simulink model "drone_yolo_simulasyon"  (R2025b)
settings: Solver=VariableStepAuto  StartTime=0.0  StopTime=15.0  RelTol=1e-3
undefined symbols (not defined in the file): Sim3dSensor
libraries: visionsources x1, pycoexlib x1, visiongeotforms x1, sim3dcameralib x1, sim3dlib x1, uavsim3dlib x1
settings Model: Creator=sario  LastModifiedBy=sario

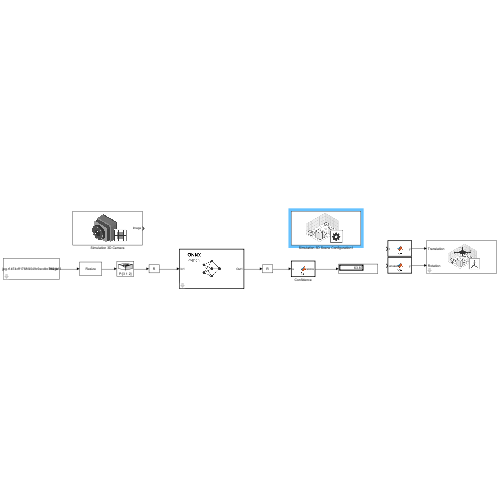
[thumbnail: Simulink's stored preview of the top-level diagram]
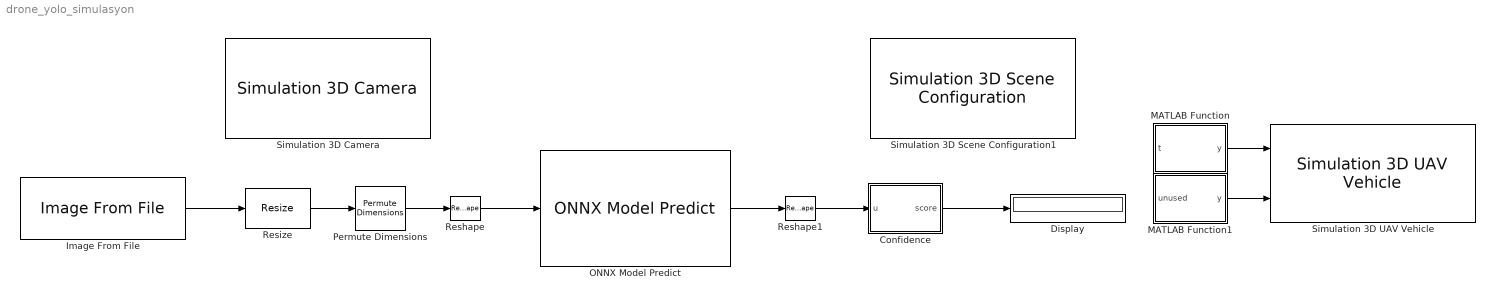
== system drone_yolo_simulasyon ==
  Confidence : MATLAB Function  TreatAsAtomicUnit=on
  Display : Display
  Image From File : visionsources/Image From File  Tag=vipblks_nd  FileName=C:\Users\sario\OneDrive\Masaüstü\crack_tespit.v1i.yolov8\test\images\00024_jpg.rf.b74cff1768f4049c9ecdbc7851b1f85d.jpg  Ts=inf  imagePorts=One multidimensional signal  OutPortLabels=R|G|B  ImageDataType=Inherit from input image  sdImageDataType=uint(8)  Signed=on  WordLength=16  FractionLengthMode=User-defined  FractionLength=15
  MATLAB Function : MATLAB Function  TreatAsAtomicUnit=on
  MATLAB Function1 : MATLAB Function  TreatAsAtomicUnit=on
  ONNX Model Predict : pycoexlib/ONNX Model Predict  ModelFile=C:\Users\sario\OneDrive\Masaüstü\crack_tespit.v1i.yolov8\best.onnx  ExecutionProviders=CPUExecutionProvider  InputTable={ 'In1', 'float32', '', '' }  OutputTable={ 'Out1', '', '' }  SampleTime=-1  InputDatatypes=float32  InputPermutations=[]  OutputPermutations=[]  PythonCoexecutionBlockType=ONNXModelBlock  VariableOutputMaxSizes=[]
  Permute Dimensions : PermuteDimensions  Order=[3 1 2]
  Reshape : Reshape  OutputDimensionality=Customize  OutputDimensions=[1, 3, 640, 640]
  Reshape1 : Reshape  OutputDimensionality=Customize  OutputDimensions=[6 8400]
  Resize : visiongeotforms/Resize  specify=Number of output rows and columns  rfactor=[200 150]  outCols=25  outRows=25  outRowsCols=[640 640]  interp_method=Bilinear  antialias=on  useROI=off  roiFlag=off  roundingMode=Nearest  overflowMode=on  prodOutputMode=Binary point scaling  prodOutputWordLength=32  prodOutputFracLength=10
  Simulation 3D Camera : sim3dcameralib/Simulation 3D Camera  Priority=1  sensorTag=Sim3dSensor�  sensorId=1  sensorName=Sim3dSensor�  vehTagList={'Scene Origin';'SimulinkVehicle1'}  vehTag=SimulinkVehicle1  CoordinateSystem=ISO8855  mountLoc=Origin  offsetFlag=on  tmountOffset=[0, 0, 0]  extTmount=off  rmountOffset=[0, 0, 0]  extRmount=off  FocalLength=[1109, 1109]  OpticalCenter=[640, 360]  ImageSize=[720, 1280]  RadialDistortion=[0, 0]  TangentialDistortion=[0, 0]  SensorSkew=0  VisualizeFieldOfView=off  FieldOfViewRange=61  DepthOutportEnabled=off  SemanticOutportEnabled=off  TransformOutportEnabled=off  SampleTime=-1  mountPoint=[0 0 0]  mountOrientation=[0 0 0]  aMode=4  ID=1
      settings: LibrarySourceBlock=uavsim3dlib/Simulation 3D Camera
  Simulation 3D Scene Configuration1 : sim3dlib/Simulation 3D Scene Configuration  Priority=0  ProjectFormat=Default Scenes  SceneDesc=US city block  ProjectName=C:\Program Files\MATLAB\R2025b\toolbox\shared\sim3d_projects\automotive_project_windows\UE\WindowsNoEditor\VehicleSimulation.exe  ScenePath=/Game/Maps/USCityBlock  EnableOpenDRIVE=off  vehTagList={'Custom';'Scene Origin';'SimulinkVehicle1'}  vehTag=SimulinkVehicle1  AttachedCameraRelativeTranslation=[0 0 0]  FreeCameraDefaultInitialTranslation=[-6, 0, 2]  AttachedCameraRelativeRotation=[0 0 0]  FreeCameraDefaultInitialRotation=[0, -15, 0]  ViewpointName=Custom  FreeCameraInitialTranslation=[0, 0, 0]  ViewpointTranslation=[0, 0, 0]  FreeCameraInitialRotation=[0, 0, 0]  ViewpointRotation=[0, 0, 0]  OpVisEn=off  Ts=1/60  EnableWindow=on  EnableRemoteAccess=off  EnableWeather=off  SunAzimuth=90  SunAltitude=40.0  EnableGeospatialSun=off  Latitude=0  Longitude=0  Date=2023-01-01  Time=10:30:00  GeoTimeZone=-5.0  SunDaylightSaving=off  wind=1  clouds=10  EnableVolumetricClouds=off  CloudCoverage=0  CloudAltitude=6  fog=0  rain=0  RaindropsEffect=off  SnowDensity=0  EnableGeospatial=off  TilesetSource=Earth terrain  UseTrueOrigin=off  OriginHeight=200  OriginLatitude=40.744652  OriginLongitude=-73.988864  MapStyle=Aerial  AdditionalAssetIDs=[]  UseAdvancedSunSky=off  SolarTime=11  TimeZone=-5  Day=21  Month=9  Year=2022  UseDaylightSavingTime=on  DSTStartDay=10  DSTStartMonth=3  DSTEndDay=3  DSTEndMonth=11  DSTSwitchHour=2  sensorTag=MainCamera2  sensorId=2  sensorName=MainCamera2  mountLoc=Origin  offsetFlag=off  tmountOffset=[0, 0, 0]  rmountOffset=[0, 0, 0]  HorizontalResolution=1280  VerticalResolution=720  HorizontalFOV=60  mountPoint=[0 0 0]  mountOrientation=[0 0 0]  aMode=4  ID=2  GeoTrigger=Inactive  ViewNameList={'Custom'}  ViewTranslationList={'[0 0 0]'}  ViewRotationList={'[0 0 0]'}
      settings: LibrarySourceBlock=uavsim3dlib/Simulation 3D Scene Configuration
  Simulation 3D UAV Vehicle : uavsim3dlib/Simulation 3D UAV Vehicle  Priority=-1  Mesh=Quadrotor  MeshPath=/MathWorksUAVContent/UAVs/HexaRotorUAV/HexaRotor.HexaRotor  Color=Black  ActorName=SimulinkVehicle1  UseGlobalFrame=off  InitialTranslation=[0 0 0]  InitialRotation=[0 0 0]  InitialTranslationGlobal=[0 0 0]  InitialGeoOrigin=[0 0 0]  InitialRotationGlobal=[0 0 0]  SampleTime=-1  ActorType=SimulinkVehicle  ID=1  aMode=4  ActorTag=SimulinkVehicle1
  wires:
  Resize/1 -> Permute Dimensions/1
  Permute Dimensions/1 -> Reshape/1
  Reshape/1 -> ONNX Model Predict/1
  MATLAB Function/1(y) -> Simulation 3D UAV Vehicle/1
  MATLAB Function1/1(y) -> Simulation 3D UAV Vehicle/2
  Image From File/1 -> Resize/1
  ONNX Model Predict/1 -> Reshape1/1
  Reshape1/1 -> Confidence/1(u)
  Confidence/1(score) -> Display/1

== matlab function drone_yolo_simulasyon/MATLAB Function ==
  data: y output; t input
function y = fcn(t)
% y = [x; y; z]

x = 0.2 * t;      % İleri doğru hareket
y_pos = 0;        % Sağa-sola hareket yok
z = 15;           % 15 metre yükseklik

y = [x; y_pos; z];
end

== matlab function drone_yolo_simulasyon/Confidence ==
  data: u input; score output
function score = fcn(u)
v = u(:);
m = max(v);
score = m / single(10);
end

== matlab function drone_yolo_simulasyon/MATLAB Function1 ==
  data: y output; unused input
function y = fcn(~)
% [roll; pitch; yaw]
y = [0; 0; 0];
end
